simulink model "ZT_VehCtrl_18B_CAN"  (R2018b)
settings: Solver=FixedStepAuto  StartTime=0.0  StopTime=inf  FixedStep=0.005  RelTol=1e-3
InitFcn:
  | mbd_mpc_consistency_checks(bdroot(gcs));
values from neighbouring files (symbols this model uses):
  BatoverTempTh = single(80)    [VCU_INIT.m]
  BRS_PwrValid = single(5)    [VCU_INIT.m]
  BRSEnSpdTh1 = single(10)    [VCU_INIT.m]
  BRSEnSpdTh2 = single(20)    [VCU_INIT.m]
  MCUTempAlarmTh = single (60)    [VCU_INIT.m]
  mps2kmh = single(3.6)    [VCU_INIT.m]
  MtrPwrFac = single(1/9550)    [VCU_INIT.m]
  MtrTempAlarmTh = single (50)    [VCU_INIT.m]
  Padle1Signal1_Th = [PadleSignal1_min,PadleSignal1_max]    [VCU_INIT.m]
  Padle1Signal2_Th = [PadleSignal2_min,PadleSignal2_max]    [VCU_INIT.m]
  PadleSignal1_max = 3.84    [VCU_INIT.m]
  PadleSignal1_min = 0.75    [VCU_INIT.m]
  PadleSignal2_max = 1.92    [VCU_INIT.m]
  PadleSignal2_min = 0.375    [VCU_INIT.m]
  PadleValid = 0.05    [VCU_INIT.m]
  PwrLimFactor = single(0.5)    [VCU_INIT.m]
  Ratio = single(1)    [VCU_INIT.m]
  rpm2mps = single(2*pi/60 * WhlRadius/Ratio)    [VCU_INIT.m]
  SOCLowTh = single(20)    [VCU_INIT.m]
  VehPwrBackwardMax = VehPwrMax * single(0.3)    [VCU_INIT.m]
  VehPwrMax = single(MtrPwrMax * 4)    [VCU_INIT.m]
  VehTrqBackwardMax = VehTrqMax * single(0.3)    [VCU_INIT.m]
  VehTrqMax = single(MtrTrqMax * Ratio *4)    [VCU_INIT.m]
  WhlRadius = single(1)    [VCU_INIT.m]
undefined symbols (not defined in the file or in its folder): Delay_Charge, Delay_Discharge, fifo_0_vect, fifo_1_vect, LQFP, pts1_fifo_0_vect, pts1_fifo_1_vect, pts2_fifo_0_vect, pts2_fifo_1_vect, pts3_fifo_0_vect, pts3_fifo_1_vect, pts4_fifo_0_vect, pts4_fifo_1_vect
libraries: mbd_mpc574x_ec_toolbox x157, canmsglib x74, simulink x38
(part 3 of 12)

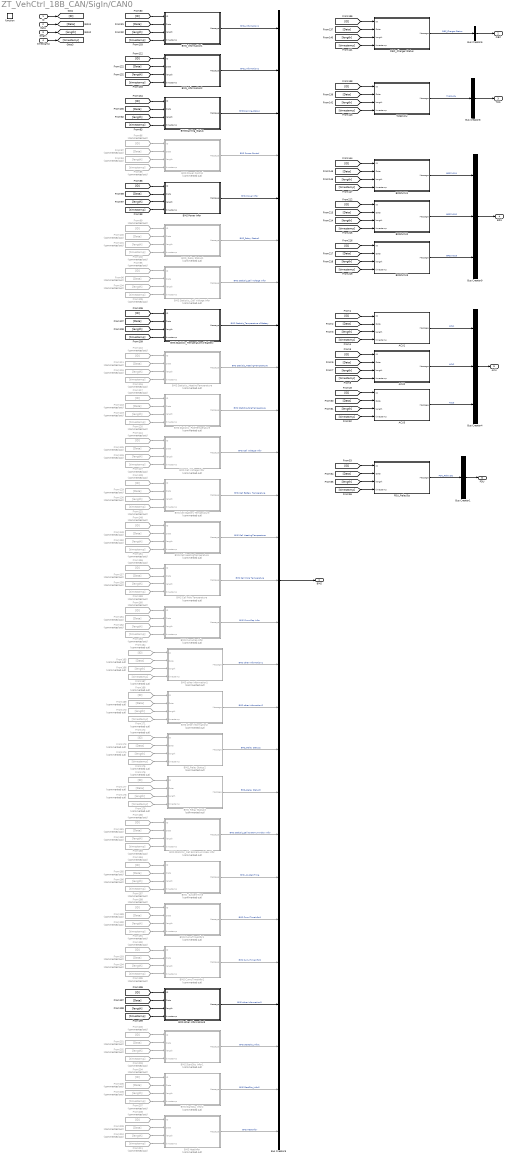
== system ZT_VehCtrl_18B_CAN/SigIn/CAN0  ==
  ID : Inport
  Data : Inport  Port=2
  length : Inport  Port=3
  timestamp : Inport  Port=4
  function : TriggerPort  TriggerType=function-call  VariantControl=Variant
  " BMS Power Control" : Subsystem  Commented=on
  ACU1 : Subsystem
  ACU2 : Subsystem
  ACU3 : Subsystem
  BMS Cell Battery Temperature : Subsystem  Commented=on
  BMS Cell HeatingTemperature : Subsystem  Commented=on
  BMS Cell Pole Temperature : Subsystem  Commented=on
  BMS Cell Voltage Infor : Subsystem  Commented=on
  BMS CumuCap Infor : Subsystem  Commented=on
  BMS CumuTimeInfor1 : Subsystem  Commented=on
  BMS CumuTimeInfor2 : Subsystem  Commented=on
  BMS HeatInfor : Subsystem  Commented=on
  BMS Power Infor : Subsystem
  BMS StartDia_Infor1 : Subsystem  Commented=on
  BMS StartDia_Infor2 : Subsystem  Commented=on
  BMS Statistic_Cell ExtremumIndex Infor : Subsystem  Commented=on
  BMS Statistic_Cell Voltage Infor : Subsystem  Commented=on
  BMS Statistic_HeatingTemperature : Subsystem  Commented=on
  BMS Statistic_PoleTemperature : Subsystem  Commented=on
  BMS Statistic_Temperature of Battery : Subsystem
  "BMS _SystemTime " : Subsystem  Commented=on
  BMS other Information1 : Subsystem  Commented=on
  "BMS other Information2 " : Subsystem  Commented=on
  BMS other Information3 : Subsystem
  BMSWarning_Status : Subsystem
  BMS_Information1 : Subsystem
  BMS_Information2 : Subsystem
  BMS_Relay Status1 : Subsystem  Commented=on
  BMS_Relay Status2 : Subsystem  Commented=on
  BMS_Relay Status3 : Subsystem  Commented=on
  BRS2VCU1 : Subsystem
  BRS2VCU2 : Subsystem
  BRS2VCU3 : Subsystem
  Bus Creator1 : BusCreator  Inputs=1
  Bus Creator4 : BusCreator  Inputs=3
  Bus Creator5 : BusCreator  Inputs=27
  Bus Creator6 : BusCreator  Inputs=1
  Bus Creator8 : BusCreator  Inputs=1
  Bus Creator9 : BusCreator  Inputs=3
  From{87,96,100,111,118,125,129,149,157,161,165,169,173,177,181,185,189,193,201,205,209} (21 alike) : From  Commented=on  GotoTag=Data
  From{84,101,104,115,119,126,130,150,158,162,166,170,174,178,182,186,190,194,202,206,210} (21 alike) : From  Commented=on  GotoTag=length
  From{85,102,105,116,120,127,131,151,159,163,167,171,175,179,183,187,191,195,203,207,211} (21 alike) : From  Commented=on  GotoTag=timestamp
  From{86,95,99,110,117,124,128,148,156,160,164,168,172,176,180,184,188,192,200,204,208} (21 alike) : From  Commented=on  GotoTag=ID
  OBC_Charger Status : Subsystem
  PDU_RelaySts : Subsystem
  TMS2VCU : Subsystem
  BMS : Outport
  OBC : Outport  Port=2
  TMS : Outport  Port=3
  "BRS " : Outport  Port=4
  ACU : Outport  Port=5
  PDU : Outport  Port=6
  wires:
  [timestamp] -> BMS Statistic_Temperature of Battery/4(timestamp)
  From128/1 -> BMS Cell Battery Temperature/1(ID)
  BMS Statistic_PoleTemperature/1(Message) -> Bus Creator5/10  "BMS Statistic_PoleTemperature"
  From100/1 -> BMS_Relay Status1/2(Data)
  BMS Statistic_Temperature of Battery/1(Message) -> Bus Creator5/8  "BMS Statistic_Temperature of Battery"
  BMS Statistic_HeatingTemperature/1(Message) -> Bus Creator5/9  "BMS Statistic_HeatingTemperature"
  From130/1 -> BMS Cell Battery Temperature/3(length)
  From105/1 -> BMS Statistic_Cell Voltage Infor/4(timestamp)
  [length] -> BMS Statistic_Temperature of Battery/3(length)
  BMS Power Infor/1(Message) -> Bus Creator5/5  "BMS Power Infor"
  From131/1 -> BMS Cell Battery Temperature/4(timestamp)
  From117/1 -> BMS Statistic_PoleTemperature/1(ID)
  BMS Cell Battery Temperature/1(Message) -> Bus Creator5/12  "BMS Cell Battery Temperature"
  From96/1 -> BMS Statistic_Cell Voltage Infor/2(Data)
  From119/1 -> BMS Statistic_PoleTemperature/3(length)
  From120/1 -> BMS Statistic_PoleTemperature/4(timestamp)
  From87/1 -> " BMS Power Control"/2(Data)
  From118/1 -> BMS Statistic_PoleTemperature/2(Data)
  From125/1 -> BMS Cell Voltage Infor/2(Data)
  BMS_Relay Status1/1(Message) -> Bus Creator5/6  "BMS_Relay Status1"
  [timestamp] -> BMSWarning_Status/4(timestamp)
  From95/1 -> BMS Statistic_Cell Voltage Infor/1(ID)
  [Data] -> BMS Statistic_Temperature of Battery/2(Data)
  [length] -> BMSWarning_Status/3(length)
  From116/1 -> BMS Statistic_HeatingTemperature/4(timestamp)
  Bus Creator5/1 -> BMS/1
  From85/1 -> " BMS Power Control"/4(timestamp)
  From111/1 -> BMS Statistic_HeatingTemperature/2(Data)
  From86/1 -> " BMS Power Control"/1(ID)
  [Data] -> BMS Power Infor/2(Data)
  BMS Statistic_Cell Voltage Infor/1(Message) -> Bus Creator5/7  "BMS Statistic_Cell Voltage Infor"
  [ID] -> BMSWarning_Status/1(ID)
  From129/1 -> BMS Cell Battery Temperature/2(Data)
  [Data] -> BMSWarning_Status/2(Data)
  From84/1 -> " BMS Power Control"/3(length)
  From124/1 -> BMS Cell Voltage Infor/1(ID)
  BMSWarning_Status/1(Message) -> Bus Creator5/3  "BMSWarning_Status"
  From127/1 -> BMS Cell Voltage Infor/4(timestamp)
  From115/1 -> BMS Statistic_HeatingTemperature/3(length)
  From102/1 -> BMS_Relay Status1/4(timestamp)
  From110/1 -> BMS Statistic_HeatingTemperature/1(ID)
  From104/1 -> BMS Statistic_Cell Voltage Infor/3(length)
  From101/1 -> BMS_Relay Status1/3(length)
  " BMS Power Control"/1(Message) -> Bus Creator5/4  "BMS Power Control"
  [ID] -> BMS Power Infor/1(ID)
  From126/1 -> BMS Cell Voltage Infor/3(length)
  [timestamp] -> BMS Power Infor/4(timestamp)
  [ID] -> BMS Statistic_Temperature of Battery/1(ID)
  BMS Cell Voltage Infor/1(Message) -> Bus Creator5/11  "BMS Cell Voltage Infor"
  From99/1 -> BMS_Relay Status1/1(ID)
  [length] -> BMS Power Infor/3(length)
  [Data] -> OBC_Charger Status/2(Data)
  OBC_Charger Status/1(Message) -> Bus Creator6/1  "OBC_Charger Status"
  [length] -> OBC_Charger Status/3(length)
  [ID] -> OBC_Charger Status/1(ID)
  Bus Creator6/1 -> OBC/1
  [timestamp] -> OBC_Charger Status/4(timestamp)
  BMS_Information2/1(Message) -> Bus Creator5/2  "BMS_Information2"
  BMS_Information1/1(Message) -> Bus Creator5/1  "BMS_Information1"
  [ID] -> BMS_Information2/1(ID)
  [Data] -> BMS_Information2/2(Data)
  [length] -> BMS_Information2/3(length)
  [timestamp] -> BMS_Information1/4(timestamp)
  [length] -> BMS_Information1/3(length)
  [Data] -> BMS_Information1/2(Data)
  [ID] -> BMS_Information1/1(ID)
  [timestamp] -> BMS_Information2/4(timestamp)
  From149/1 -> BMS Cell HeatingTemperature/2(Data)
  BMS Cell HeatingTemperature/1(Message) -> Bus Creator5/13  "BMS Cell HeatingTemperature"
  From151/1 -> BMS Cell HeatingTemperature/4(timestamp)
  From150/1 -> BMS Cell HeatingTemperature/3(length)
  From148/1 -> BMS Cell HeatingTemperature/1(ID)
  From156/1 -> BMS Cell Pole Temperature/1(ID)
  From158/1 -> BMS Cell Pole Temperature/3(length)
  From159/1 -> BMS Cell Pole Temperature/4(timestamp)
  BMS Cell Pole Temperature/1(Message) -> Bus Creator5/14  "BMS Cell Pole Temperature"
  From157/1 -> BMS Cell Pole Temperature/2(Data)
  From161/1 -> BMS CumuCap Infor/2(Data)
  BMS CumuCap Infor/1(Message) -> Bus Creator5/15  "BMS CumuCap Infor"
  From163/1 -> BMS CumuCap Infor/4(timestamp)
  From162/1 -> BMS CumuCap Infor/3(length)
  From160/1 -> BMS CumuCap Infor/1(ID)
  From164/1 -> BMS other Information1/1(ID)
  From166/1 -> BMS other Information1/3(length)
  From167/1 -> BMS other Information1/4(timestamp)
  BMS other Information1/1(Message) -> Bus Creator5/16  "BMS other Information1"
  From165/1 -> BMS other Information1/2(Data)
  From169/1 -> "BMS other Information2 "/2(Data)
  "BMS other Information2 "/1(Message) -> Bus Creator5/17  "BMS other Information2"
  From171/1 -> "BMS other Information2 "/4(timestamp)
  From170/1 -> "BMS other Information2 "/3(length)
  From168/1 -> "BMS other Information2 "/1(ID)
  From172/1 -> BMS_Relay Status2/1(ID)
  From174/1 -> BMS_Relay Status2/3(length)
  From175/1 -> BMS_Relay Status2/4(timestamp)
  BMS_Relay Status2/1(Message) -> Bus Creator5/18  "BMS_Relay Status2"
  From173/1 -> BMS_Relay Status2/2(Data)
  From177/1 -> BMS_Relay Status3/2(Data)
  BMS_Relay Status3/1(Message) -> Bus Creator5/19  "BMS_Relay Status3"
  From179/1 -> BMS_Relay Status3/4(timestamp)
  From178/1 -> BMS_Relay Status3/3(length)
  From176/1 -> BMS_Relay Status3/1(ID)
  From180/1 -> BMS Statistic_Cell ExtremumIndex Infor/1(ID)
  From182/1 -> BMS Statistic_Cell ExtremumIndex Infor/3(length)
  From183/1 -> BMS Statistic_Cell ExtremumIndex Infor/4(timestamp)
  BMS Statistic_Cell ExtremumIndex Infor/1(Message) -> Bus Creator5/20  "BMS Statistic_Cell ExtremumIndex Infor"
  From181/1 -> BMS Statistic_Cell ExtremumIndex Infor/2(Data)
  From185/1 -> "BMS _SystemTime "/2(Data)
  "BMS _SystemTime "/1(Message) -> Bus Creator5/21  "BMS _SystemTime"
  From187/1 -> "BMS _SystemTime "/4(timestamp)
  From186/1 -> "BMS _SystemTime "/3(length)
  From184/1 -> "BMS _SystemTime "/1(ID)
  From188/1 -> BMS CumuTimeInfor1/1(ID)
  From190/1 -> BMS CumuTimeInfor1/3(length)
  From191/1 -> BMS CumuTimeInfor1/4(timestamp)
  BMS CumuTimeInfor1/1(Message) -> Bus Creator5/22  "BMS CumuTimeInfor1"
  From189/1 -> BMS CumuTimeInfor1/2(Data)
  From193/1 -> BMS CumuTimeInfor2/2(Data)
  BMS CumuTimeInfor2/1(Message) -> Bus Creator5/23  "BMS CumuTimeInfor2"
  From195/1 -> BMS CumuTimeInfor2/4(timestamp)
  From194/1 -> BMS CumuTimeInfor2/3(length)
  From192/1 -> BMS CumuTimeInfor2/1(ID)
  [ID] -> BMS other Information3/1(ID)
  [length] -> BMS other Information3/3(length)
  [timestamp] -> BMS other Information3/4(timestamp)
  BMS other Information3/1(Message) -> Bus Creator5/24  "BMS other Information3"
  [Data] -> BMS other Information3/2(Data)
  From201/1 -> BMS StartDia_Infor1/2(Data)
  BMS StartDia_Infor1/1(Message) -> Bus Creator5/25  "BMS StartDia_Infor1"
  From203/1 -> BMS StartDia_Infor1/4(timestamp)
  From202/1 -> BMS StartDia_Infor1/3(length)
  From200/1 -> BMS StartDia_Infor1/1(ID)
  From204/1 -> BMS StartDia_Infor2/1(ID)
  From206/1 -> BMS StartDia_Infor2/3(length)
  From207/1 -> BMS StartDia_Infor2/4(timestamp)
  BMS StartDia_Infor2/1(Message) -> Bus Creator5/26  "BMS StartDia_Infor2"
  From205/1 -> BMS StartDia_Infor2/2(Data)
  From209/1 -> BMS HeatInfor/2(Data)
  BMS HeatInfor/1(Message) -> Bus Creator5/27  "BMS HeatInfor"
  From211/1 -> BMS HeatInfor/4(timestamp)
  From210/1 -> BMS HeatInfor/3(length)
  From208/1 -> BMS HeatInfor/1(ID)
  [timestamp] -> TMS2VCU/4(timestamp)
  Bus Creator8/1 -> TMS/1
  [ID] -> TMS2VCU/1(ID)
  [length] -> TMS2VCU/3(length)
  TMS2VCU/1(Message) -> Bus Creator8/1  "TMS2VCU"
  [Data] -> TMS2VCU/2(Data)
  [Data] -> BRS2VCU1/2(Data)
  BRS2VCU1/1(Message) -> Bus Creator9/1  "BRS2VCU1"
  [length] -> BRS2VCU1/3(length)
  [ID] -> BRS2VCU1/1(ID)
  Bus Creator9/1 -> "BRS "/1
  [timestamp] -> BRS2VCU1/4(timestamp)
  [timestamp] -> BRS2VCU2/4(timestamp)
  [ID] -> BRS2VCU2/1(ID)
  [length] -> BRS2VCU2/3(length)
  [Data] -> BRS2VCU2/2(Data)
  [Data] -> BRS2VCU3/2(Data)
  [length] -> BRS2VCU3/3(length)
  [ID] -> BRS2VCU3/1(ID)
  [timestamp] -> BRS2VCU3/4(timestamp)
  BRS2VCU2/1(Message) -> Bus Creator9/2  "BRS2VCU2"
  BRS2VCU3/1(Message) -> Bus Creator9/3  "BRS2VCU3"
  length/1 -> [length]
  ID/1 -> [ID]
  timestamp/1 -> [timestamp]
  Data/1 -> [Data]
  [Data] -> ACU1/2(Data)
  [timestamp] -> ACU1/4(timestamp)
  [length] -> ACU2/3(length)
  [timestamp] -> ACU3/4(timestamp)
  [ID] -> ACU3/1(ID)
  ACU2/1(Message) -> Bus Creator4/2  "ACU2"
  Bus Creator4/1 -> ACU/1
  [Data] -> ACU2/2(Data)
  [length] -> ACU1/3(length)
  [timestamp] -> ACU2/4(timestamp)
  [ID] -> ACU1/1(ID)
  [length] -> ACU3/3(length)
  ACU1/1(Message) -> Bus Creator4/1  "ACU1"
  ACU3/1(Message) -> Bus Creator4/3  "ACU3"
  [Data] -> ACU3/2(Data)
  [ID] -> ACU2/1(ID)
  Bus Creator1/1 -> PDU/1
  [length] -> PDU_RelaySts/3(length)
  PDU_RelaySts/1(Message) -> Bus Creator1/1  "PDU_RelaySts"
  [Data] -> PDU_RelaySts/2(Data)
  [timestamp] -> PDU_RelaySts/4(timestamp)
  [ID] -> PDU_RelaySts/1(ID)

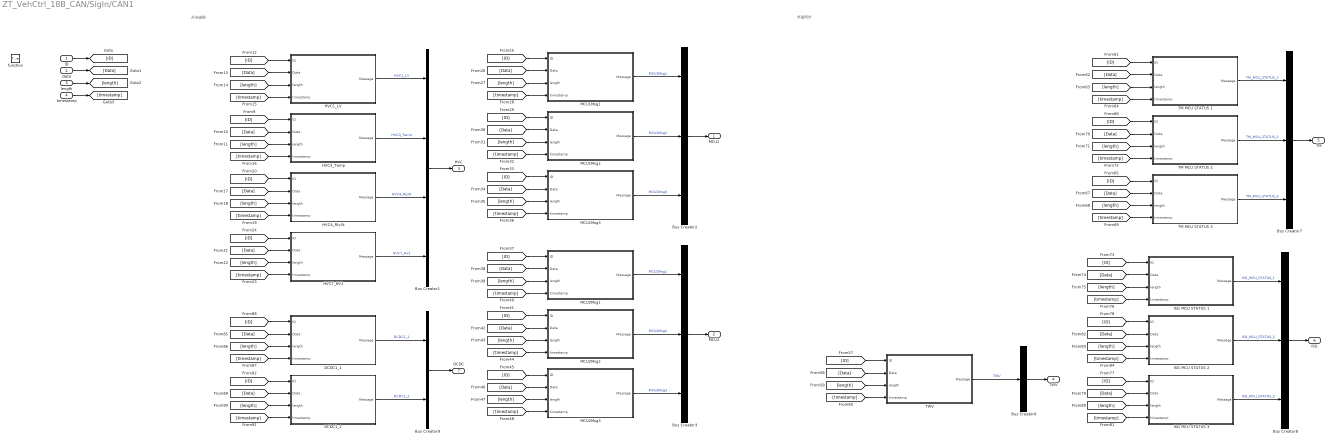
== system ZT_VehCtrl_18B_CAN/SigIn/CAN1 ==
  note: 永磁同步
  note: 开关磁阻
  ID : Inport
  Data : Inport  Port=2
  length : Inport  Port=3
  timestamp : Inport  Port=4
  function : TriggerPort  TriggerType=function-call  VariantControl=Variant
  Bus Creator1 : BusCreator  Inputs=4
  Bus Creator{2..3,7..8} (4 alike) : BusCreator  Inputs=3
  Bus Creator6 : BusCreator  Inputs=1
  Bus Creator9 : BusCreator  Inputs=2
  DCDC1_1 : Subsystem
  DCDC1_2 : Subsystem
  HVC1_LV : Subsystem
  HVC3_Temp : Subsystem
  HVC4_RlySt : Subsystem
  HVC7_HV1 : Subsystem
  ISG MCU STATUS 1 : Subsystem
  ISG MCU STATUS 2 : Subsystem
  ISG MCU STATUS 3 : Subsystem
  MCU1Msg1 : Subsystem
  MCU1Msg2 : Subsystem
  MCU1Msg3 : Subsystem
  MCU2Msg1 : Subsystem
  MCU2Msg2 : Subsystem
  MCU2Msg3 : Subsystem
  TM MCU STATUS 1 : Subsystem
  TM MCU STATUS 2 : Subsystem
  TM MCU STATUS 3 : Subsystem
  "TWV " : Subsystem
  MCU1 : Outport
  MCU2 : Outport  Port=2
  HVC : Outport  Port=3
  TWV : Outport  Port=4
  TM : Outport  Port=5
  "ISG " : Outport  Port=6
  DCDC : Outport  Port=7
  wires:
  length/1 -> [length]
  timestamp/1 -> [timestamp]
  Data/1 -> [Data]
  ID/1 -> [ID]
  Bus Creator2/1 -> MCU1/1
  [Data] -> HVC1_LV/2(Data)
  [timestamp] -> HVC1_LV/4(timestamp)
  [ID] -> HVC1_LV/1(ID)
  HVC1_LV/1(Message) -> Bus Creator1/1  "HVC1_LV"
  [length] -> HVC1_LV/3(length)
  [length] -> HVC3_Temp/3(length)
  HVC3_Temp/1(Message) -> Bus Creator1/2  "HVC3_Temp"
  [ID] -> HVC3_Temp/1(ID)
  [timestamp] -> HVC3_Temp/4(timestamp)
  [Data] -> HVC3_Temp/2(Data)
  [Data] -> HVC4_RlySt/2(Data)
  [timestamp] -> HVC4_RlySt/4(timestamp)
  [ID] -> HVC4_RlySt/1(ID)
  [length] -> HVC4_RlySt/3(length)
  HVC4_RlySt/1(Message) -> Bus Creator1/3  "HVC4_RlySt"
  HVC7_HV1/1(Message) -> Bus Creator1/4  "HVC7_HV1"
  [length] -> HVC7_HV1/3(length)
  [ID] -> HVC7_HV1/1(ID)
  [timestamp] -> HVC7_HV1/4(timestamp)
  [Data] -> HVC7_HV1/2(Data)
  [length] -> MCU1Msg1/3(length)
  MCU1Msg1/1(Message) -> Bus Creator2/1  "MCU1Msg1"
  [ID] -> MCU1Msg1/1(ID)
  [timestamp] -> MCU1Msg1/4(timestamp)
  [Data] -> MCU1Msg1/2(Data)
  [Data] -> MCU1Msg2/2(Data)
  [timestamp] -> MCU1Msg2/4(timestamp)
  [ID] -> MCU1Msg2/1(ID)
  MCU1Msg2/1(Message) -> Bus Creator2/2  "MCU1Msg2"
  [length] -> MCU1Msg2/3(length)
  [length] -> MCU1Msg3/3(length)
  [ID] -> MCU1Msg3/1(ID)
  [timestamp] -> MCU1Msg3/4(timestamp)
  [Data] -> MCU1Msg3/2(Data)
  MCU1Msg3/1(Message) -> Bus Creator2/3  "MCU1Msg3"
  MCU2Msg3/1(Message) -> Bus Creator3/3  "MCU2Msg3"
  [Data] -> MCU2Msg3/2(Data)
  [timestamp] -> MCU2Msg3/4(timestamp)
  [ID] -> MCU2Msg3/1(ID)
  [length] -> MCU2Msg3/3(length)
  [length] -> MCU2Msg2/3(length)
  MCU2Msg2/1(Message) -> Bus Creator3/2  "MCU2Msg2"
  [ID] -> MCU2Msg2/1(ID)
  [timestamp] -> MCU2Msg2/4(timestamp)
  [Data] -> MCU2Msg2/2(Data)
  [Data] -> MCU2Msg1/2(Data)
  [timestamp] -> MCU2Msg1/4(timestamp)
  [ID] -> MCU2Msg1/1(ID)
  MCU2Msg1/1(Message) -> Bus Creator3/1  "MCU2Msg1"
  [length] -> MCU2Msg1/3(length)
  Bus Creator6/1 -> TWV/1
  "TWV "/1(Message) -> Bus Creator6/1  "TWV"
  [Data] -> "TWV "/2(Data)
  [timestamp] -> "TWV "/4(timestamp)
  [ID] -> "TWV "/1(ID)
  [length] -> "TWV "/3(length)
  Bus Creator7/1 -> TM/1
  [length] -> TM MCU STATUS 1/3(length)
  TM MCU STATUS 1/1(Message) -> Bus Creator7/1  "TM_MCU_STATUS_1"
  [ID] -> TM MCU STATUS 1/1(ID)
  [timestamp] -> TM MCU STATUS 1/4(timestamp)
  [Data] -> TM MCU STATUS 1/2(Data)
  [Data] -> TM MCU STATUS 2/2(Data)
  [timestamp] -> TM MCU STATUS 2/4(timestamp)
  [ID] -> TM MCU STATUS 2/1(ID)
  TM MCU STATUS 2/1(Message) -> Bus Creator7/2  "TM_MCU_STATUS_2"
  [length] -> TM MCU STATUS 2/3(length)
  [length] -> TM MCU STATUS 3/3(length)
  [ID] -> TM MCU STATUS 3/1(ID)
  [timestamp] -> TM MCU STATUS 3/4(timestamp)
  [Data] -> TM MCU STATUS 3/2(Data)
  TM MCU STATUS 3/1(Message) -> Bus Creator7/3  "TM_MCU_STATUS_3"
  ISG MCU STATUS 3/1(Message) -> Bus Creator8/3  "ISG_MCU_STATUS_3"
  [Data] -> ISG MCU STATUS 3/2(Data)
  [timestamp] -> ISG MCU STATUS 3/4(timestamp)
  [ID] -> ISG MCU STATUS 3/1(ID)
  [length] -> ISG MCU STATUS 3/3(length)
  [length] -> ISG MCU STATUS 2/3(length)
  ISG MCU STATUS 2/1(Message) -> Bus Creator8/2  "ISG_MCU_STATUS_2"
  [ID] -> ISG MCU STATUS 2/1(ID)
  [timestamp] -> ISG MCU STATUS 2/4(timestamp)
  [Data] -> ISG MCU STATUS 2/2(Data)
  [Data] -> ISG MCU STATUS 1/2(Data)
  [timestamp] -> ISG MCU STATUS 1/4(timestamp)
  [ID] -> ISG MCU STATUS 1/1(ID)
  ISG MCU STATUS 1/1(Message) -> Bus Creator8/1  "ISG_MCU_STATUS_1"
  [length] -> ISG MCU STATUS 1/3(length)
  Bus Creator8/1 -> "ISG "/1
  Bus Creator1/1 -> HVC/1
  Bus Creator3/1 -> MCU2/1
  [Data] -> DCDC1_2/2(Data)
  [timestamp] -> DCDC1_2/4(timestamp)
  [ID] -> DCDC1_2/1(ID)
  [length] -> DCDC1_2/3(length)
  DCDC1_2/1(Message) -> Bus Creator9/2  "DCDC1_2"
  DCDC1_1/1(Message) -> Bus Creator9/1  "DCDC1_1"
  [length] -> DCDC1_1/3(length)
  [ID] -> DCDC1_1/1(ID)
  [timestamp] -> DCDC1_1/4(timestamp)
  [Data] -> DCDC1_1/2(Data)
  Bus Creator9/1 -> DCDC/1

== system ZT_VehCtrl_18B_CAN/SigIn/DI ==
  note: DI PULLDOWN
  note: DI PULLUP
  Bus Creator : BusCreator  Inputs=14
  DI01 : mbd_mpc574x_ec_toolbox/GPIO Blocks/Digital_Input  gpio_pin=PTG5: [SIUL2_GPIO101 | General Purpose IO PG[5]]  pull_resistor=None
  DI02 : mbd_mpc574x_ec_toolbox/GPIO Blocks/Digital_Input  gpio_pin=PTG9: [SIUL2_GPIO105 | General Purpose IO PG[9]]  pull_resistor=None
  DI03 : mbd_mpc574x_ec_toolbox/GPIO Blocks/Digital_Input  gpio_pin=PTC11: [SIUL2_GPIO43 | General Purpose IO PC[11]]  pull_resistor=None
  DI04 : mbd_mpc574x_ec_toolbox/GPIO Blocks/Digital_Input  gpio_pin=PTA9: [SIUL2_GPIO9 | General Purpose IO PA[9]]  pull_resistor=None
  DI07 : mbd_mpc574x_ec_toolbox/GPIO Blocks/Digital_Input  gpio_pin=PTA0: [SIUL2_GPIO0 | General Purpose IO PA[0]]  pull_resistor=None
  DI08 : mbd_mpc574x_ec_toolbox/GPIO Blocks/Digital_Input  gpio_pin=PTD11: [SIUL2_GPIO59 | General Purpose IO PD[11]]  pull_resistor=None
  DI09 : mbd_mpc574x_ec_toolbox/GPIO Blocks/Digital_Input  gpio_pin=PTG6: [SIUL2_GPIO102 | General Purpose IO PG[6]]  pull_resistor=None
  DI10 : mbd_mpc574x_ec_toolbox/GPIO Blocks/Digital_Input  gpio_pin=PTG2: [SIUL2_GPIO98 | General Purpose IO PG[2]]  pull_resistor=None
  DI12 : mbd_mpc574x_ec_toolbox/GPIO Blocks/Digital_Input  gpio_pin=PTF13: [SIUL2_GPIO93 | General Purpose IO PF[13]]  pull_resistor=None
  DI13 : mbd_mpc574x_ec_toolbox/GPIO Blocks/Digital_Input  gpio_pin=PTG4: [SIUL2_GPIO100 | General Purpose IO PG[4]]  pull_resistor=None
  DI15 : mbd_mpc574x_ec_toolbox/GPIO Blocks/Digital_Input  gpio_pin=PTF12: [SIUL2_GPIO92 | General Purpose IO PF[12]]  pull_resistor=None
  DI16 : mbd_mpc574x_ec_toolbox/GPIO Blocks/Digital_Input  gpio_pin=PTG7: [SIUL2_GPIO103 | General Purpose IO PG[7]]  pull_resistor=None
  DI17 : mbd_mpc574x_ec_toolbox/GPIO Blocks/Digital_Input  gpio_pin=PTD10: [SIUL2_GPIO58 | General Purpose IO PD[10]]  pull_resistor=None
  DI18 : mbd_mpc574x_ec_toolbox/GPIO Blocks/Digital_Input  gpio_pin=PTG10: [SIUL2_GPIO106 | General Purpose IO PG[10]]  pull_resistor=None
  DI_31_32_33_34 : Subsystem
  Data Store Read : DataStoreRead  DataStoreName=DI07
  Data Store Read1 : DataStoreRead  DataStoreName=DI10
  Data Store Read10 : DataStoreRead  DataStoreName=DI04
  Data Store Read11 : DataStoreRead  DataStoreName=DI12
  Data Store Read12 : DataStoreRead  DataStoreName=DI08
  Data Store Read13 : DataStoreRead  DataStoreName=DI09
  Data Store Read2 : DataStoreRead  DataStoreName=DI13
  Data Store Read3 : DataStoreRead  DataStoreName=DI15
  Data Store Read4 : DataStoreRead  DataStoreName=DI16
  Data Store Read5 : DataStoreRead  DataStoreName=DI17
  Data Store Read6 : DataStoreRead  DataStoreName=DI18
  Data Store Read7 : DataStoreRead  DataStoreName=DI01
  Data Store Read8 : DataStoreRead  DataStoreName=DI02
  Data Store Read9 : DataStoreRead  DataStoreName=DI03
  Data Store Write : DataStoreWrite  DataStoreName=DI07
  Data Store Write1 : DataStoreWrite  DataStoreName=DI01
  Data Store Write10 : DataStoreWrite  DataStoreName=DI04
  Data Store Write11 : DataStoreWrite  DataStoreName=DI12
  Data Store Write12 : DataStoreWrite  DataStoreName=DI08
  Data Store Write13 : DataStoreWrite  DataStoreName=DI09
  Data Store Write2 : DataStoreWrite  DataStoreName=DI10
  Data Store Write3 : DataStoreWrite  DataStoreName=DI13
  Data Store Write4 : DataStoreWrite  DataStoreName=DI15
  Data Store Write5 : DataStoreWrite  DataStoreName=DI16
  Data Store Write6 : DataStoreWrite  DataStoreName=DI17
  Data Store Write7 : DataStoreWrite  DataStoreName=DI18
  Data Store Write8 : DataStoreWrite  DataStoreName=DI02
  Data Store Write9 : DataStoreWrite  DataStoreName=DI03
  DI : Outport
  wires:
  DI07/1 -> Data Store Write/1
  DI01/1 -> Data Store Write1/1
  DI10/1 -> Data Store Write2/1
  DI13/1 -> Data Store Write3/1
  DI15/1 -> Data Store Write4/1
  DI17/1 -> Data Store Write6/1
  DI16/1 -> Data Store Write5/1
  DI18/1 -> Data Store Write7/1
  DI09/1 -> Data Store Write13/1
  DI08/1 -> Data Store Write12/1
  DI12/1 -> Data Store Write11/1
  DI04/1 -> Data Store Write10/1
  DI02/1 -> Data Store Write8/1
  DI03/1 -> Data Store Write9/1
  Data Store Read/1 -> Bus Creator/1  "DI07"
  Data Store Read1/1 -> Bus Creator/2  "DI10"
  Data Store Read2/1 -> Bus Creator/3  "DI13"
  Data Store Read3/1 -> Bus Creator/4  "DI15"
  Data Store Read4/1 -> Bus Creator/5  "DI16"
  Data Store Read5/1 -> Bus Creator/6  "DI17"
  Data Store Read6/1 -> Bus Creator/7  "DI18"
  Data Store Read7/1 -> Bus Creator/8  "DI01"
  Data Store Read8/1 -> Bus Creator/9  "DI02"
  Data Store Read9/1 -> Bus Creator/10  "DI03"
  Data Store Read10/1 -> Bus Creator/11  "DI04"
  Data Store Read11/1 -> Bus Creator/12  "DI12"
  Data Store Read12/1 -> Bus Creator/13  "DI08"
  Data Store Read13/1 -> Bus Creator/14  "DI09"
  Bus Creator/1 -> DI/1

== system ZT_VehCtrl_18B_CAN/SigIn/PWM ==
  note: DI PWM PULLDOWN
  note: DI PWM PULLUP
  Bus Creator : BusCreator  Inputs=8
  Data Store Read : DataStoreRead  DataStoreName=DI31_PWM_DC
  Data Store Read1 : DataStoreRead  DataStoreName=DI31_PWM_FRQ
  Data Store Read2 : DataStoreRead  DataStoreName=DI32_PWM_DC
  Data Store Read3 : DataStoreRead  DataStoreName=DI32_PWM_FRQ
  Data Store Read4 : DataStoreRead  DataStoreName=DI33_PWM_DC
  Data Store Read5 : DataStoreRead  DataStoreName=DI33_PWM_FRQ
  Data Store Read6 : DataStoreRead  DataStoreName=DI34_PWM_DC
  Data Store Read7 : DataStoreRead  DataStoreName=DI34_PWM_FRQ
  Data Store Write : DataStoreWrite  DataStoreName=DI31_PWM_DC
  Data Store Write1 : DataStoreWrite  DataStoreName=DI31_PWM_FRQ
  Data Store Write2 : DataStoreWrite  DataStoreName=DI32_PWM_DC
  Data Store Write3 : DataStoreWrite  DataStoreName=DI32_PWM_FRQ
  Data Store Write4 : DataStoreWrite  DataStoreName=DI33_PWM_DC
  Data Store Write5 : DataStoreWrite  DataStoreName=DI33_PWM_FRQ
  Data Store Write6 : DataStoreWrite  DataStoreName=DI34_PWM_FRQ
  Data Store Write7 : DataStoreWrite  DataStoreName=DI34_PWM_DC
  PWM_PTS1 : Subsystem
  PWM_PTS2 : Subsystem
  PWM_PTS3 : Subsystem
  PWM_PTS4 : Subsystem
  Subsystem : Subsystem  Commented=on
  eTimer_Arm_Capture : mbd_mpc574x_ec_toolbox/Motor Control Blocks/eTIMER Blocks/eTimer_Arm_Capture  etimerModule=0  etimerChannel=2  etimerArmAction=Start
  eTimer_Arm_Capture1 : mbd_mpc574x_ec_toolbox/Motor Control Blocks/eTIMER Blocks/eTimer_Arm_Capture  etimerModule=1  etimerChannel=2  etimerArmAction=Start
  eTimer_Arm_Capture2 : mbd_mpc574x_ec_toolbox/Motor Control Blocks/eTIMER Blocks/eTimer_Arm_Capture  etimerModule=1  etimerChannel=1  etimerArmAction=Start
  eTimer_Arm_Capture3 : mbd_mpc574x_ec_toolbox/Motor Control Blocks/eTIMER Blocks/eTimer_Arm_Capture  etimerModule=1  etimerChannel=3  etimerArmAction=Start
  PWMIn : Outport
  wires:
  Bus Creator/1 -> PWMIn/1
  Data Store Read7/1 -> Bus Creator/8  "DI34_PWM_FRQ"
  Data Store Read6/1 -> Bus Creator/7  "DI34_PWM_DC"
  Data Store Read5/1 -> Bus Creator/6  "DI33_PWM_FRQ"
  Data Store Read4/1 -> Bus Creator/5  "DI33_PWM_DC"
  Data Store Read3/1 -> Bus Creator/4  "DI32_PWM_FRQ"
  Data Store Read2/1 -> Bus Creator/3  "DI32_PWM_DC"
  Data Store Read1/1 -> Bus Creator/2  "DI31_PWM_FRQ"
  Data Store Read/1 -> Bus Creator/1  "DI31_PWM_DC"
  PWM_PTS4/1(DC) -> Data Store Write/1
  PWM_PTS4/2(freq) -> Data Store Write1/1
  PWM_PTS1/1(DC) -> Data Store Write2/1
  PWM_PTS1/2(freq) -> Data Store Write3/1
  PWM_PTS2/1(DC) -> Data Store Write4/1
  PWM_PTS2/2(freq) -> Data Store Write5/1
  PWM_PTS3/2(freq) -> Data Store Write6/1
  PWM_PTS3/1(DC) -> Data Store Write7/1

== system ZT_VehCtrl_18B_CAN/SigIn/Subsystem ==
  AI08 : Inport
  AI12 : Inport  Port=2
  1-D Lookup Table : Lookup_n-D  NumberOfTableDimensions=1  BreakpointsForDimension1=Padle1Signal1_Th  Table=[0,1]  InternalRulePriority=Speed  RndMeth=Simplest  InputSameDT=on
  1-D Lookup Table1 : Lookup_n-D  NumberOfTableDimensions=1  BreakpointsForDimension1=Padle1Signal2_Th  Table=[0,1]  InternalRulePriority=Speed  RndMeth=Simplest  InputSameDT=on
  Abs : Abs
  Compare To Constant : simulink/Logic and Bit Operations/Compare To Constant  relop=<=  const=PadleValid  OutDataTypeStr=boolean
  Constant2 : Constant  Value=0  OutDataTypeStr=single
  Data Type Conversion : DataTypeConversion  OutDataTypeStr=single
  Data Type Conversion1 : DataTypeConversion  OutDataTypeStr=single
  Saturation : Saturate  UpperLimit=PadleSignal1_max  LowerLimit=PadleSignal1_min
  Saturation1 : Saturate  UpperLimit=PadleSignal2_max  LowerLimit=PadleSignal2_min  LinearizeAsGain=off
  Subtract : Sum  Inputs=+-
  Switch : Switch  Criteria=u2 > Threshold
  "ACCPadle " : Outport
  wires:
  Subtract/1 -> Abs/1
  Saturation/1 -> 1-D Lookup Table/1
  Saturation1/1 -> 1-D Lookup Table1/1
  1-D Lookup Table/1 -> Data Type Conversion/1, Subtract/1
  Switch/1 -> Data Type Conversion1/1
  Constant2/1 -> Switch/3
  1-D Lookup Table1/1 -> Subtract/2
  Data Type Conversion/1 -> Switch/1
  Compare To Constant/1 -> Switch/2
  Abs/1 -> Compare To Constant/1
  AI08/1 -> Saturation/1
  AI12/1 -> Saturation1/1
  Data Type Conversion1/1 -> "ACCPadle "/1

== system ZT_VehCtrl_18B_CAN/SigOut/ACU ==
  "ACU_OUT " : Inport
  Trigger : TriggerPort  VariantControl=Variant  PortDimensions=1
  Add : Sum
  Bus Selector : BusSelector  OutputSignals=Data,Length
  Bus Selector1 : BusSelector  Commented=on  OutputSignals=DcacEpsCmd,DcdcCmd
  Constant : Constant  OutDataTypeStr=uint8
  Constant1 : Constant  Commented=on  Value=85
  Constant2 : Constant  Commented=on  Value=170
  Data Store Read : DataStoreRead  DataStoreName=Cnt_ACU_OUT
  Data Store Read1 : DataStoreRead  DataStoreName=DcdcCmd
  Data Store Read2 : DataStoreRead  DataStoreName=DcacEpsCmd
  Data Store Read3 : DataStoreRead  DataStoreName=DcacEpsMode
  Data Store Read4 : DataStoreRead  DataStoreName=DcacAcCmd
  Data Store Write : DataStoreWrite  DataStoreName=Cnt_ACU_OUT
  Data Type Conversion{,1..3} (4 alike) : DataTypeConversion  OutDataTypeStr=single
  FCAN_Send_ID_0x0C079AA7 : mbd_mpc574x_ec_toolbox/Communication Blocks/CAN Blocks/FCAN_Send  Priority=2  can_instance=0  can_mode=Non-blocking  can_timeout_ms=0  can_mb_idx=51  can_extended_id=on  can_is_remote=off  can_id=0C079AA7  show_adv_opts=off  can_fd_enable=off  can_enable_brs=off  can_fd_padding=0
      settings: SourceProductName=NXP Model-Based Design Toolbox for MPC57xx MCUs
  Subsystem1 : Subsystem
  Subsystem2 : Subsystem
  Subsystem3 : Subsystem
  Subsystem4 : Subsystem
  VCU_ACU1 : canmsglib/CAN Pack  CANdbFile=D:\VCU\VCU_SL_ZhengZhou\ZT2\模型与接口\CAN_DBC\动力CANB_GBK.dbc  MsgList=(none)  MsgName=VCU_ACU1  MsgIDType=Extended (29-bit identifier)  MsgIdentifier=201824935  MsgLength=8  SignalInfo=DcacAcCmd$32$8$1$2$1$0$1$0$-Inf$Inf$#DcacEpsCmd$16$8$1$2$1$0$1$0$-Inf$Inf$#DcacEpsMode$24$8$1$2$1$0$1$0$-Inf$Inf$#DcdcCmd$0$8$1$2$1$0$1$0$-Inf$Inf$#  NSignals=4  StartBits=str2num('[int32(32);int32(16);int32(24);int32(0)]')  SignalSizes=str2num('[int32(8);int32(8);int32(8);int32(8)]')  ByteOrders=str2num('[int32(1);int32(1);int32(1);int32(1)]')  DataTypes=str2num('[int32(2);int32(2);int32(2);int32(2)]')  MultiplexTypes=str2num('[int32(1);int32(1);int32(1);int32(1)]')  MultiplexValues=str2num('[double(0);double(0);double(0);double(0)]')  Factors=str2num('[double(1);double(1);double(1);double(1)]')  Offsets=str2num('[double(0);double(0);double(0);double(0)]')  Minimums=str2num('[double(-Inf);double(-Inf);double(-Inf);double(-Inf)]')  Maximums=str2num('[double(Inf);double(Inf);double(Inf);double(Inf)]')  Remote=off  ApplyMinMax=off  BusOutput=on
      settings: SourceProductName=Simulink Real-Time  SourceProductBaseCode=XP  DataFormat=CANdb specified signals
  wires:
  VCU_ACU1/1 -> Bus Selector/1
  Bus Selector/2 -> FCAN_Send_ID_0x0C079AA7/2  "<Length>"
  Bus Selector/1 -> FCAN_Send_ID_0x0C079AA7/1  "<Data>"
  Add/1 -> Data Store Write/1
  Data Store Read/1 -> Add/1
  Constant/1 -> Add/2
  "ACU_OUT "/1 -> Bus Selector1/1
  Bus Selector1/1 -> ?  "<DcacEpsCmd>"
  Bus Selector1/2 -> ?  "<DcdcCmd>"
  Subsystem1/1(Out1) -> Data Type Conversion/1
  Subsystem3/1(Out1) -> Data Type Conversion2/1
  Constant1/1 -> ?
  Constant2/1 -> ?
  Data Store Read1/1 -> Subsystem1/1(<DcacEpsCmd>)
  Data Store Read3/1 -> Subsystem2/1(<DcacEpsCmd>)
  Data Store Read2/1 -> Subsystem3/1(<DcacEpsCmd>)
  Data Store Read4/1 -> Subsystem4/1(<DcacEpsCmd>)
  Subsystem2/1(Out1) -> Data Type Conversion1/1
  Subsystem4/1(Out1) -> Data Type Conversion3/1
  Data Type Conversion/1 -> VCU_ACU1/4
  Data Type Conversion1/1 -> VCU_ACU1/3
  Data Type Conversion2/1 -> VCU_ACU1/2
  Data Type Conversion3/1 -> VCU_ACU1/1

== system ZT_VehCtrl_18B_CAN/SigOut/BMS ==
  "BMS_OUT " : Inport
  Trigger : TriggerPort  VariantControl=Variant  PortDimensions=1
  Add : Sum
  Bus Selector : BusSelector  OutputSignals=Data,Length
  Bus Selector1 : BusSelector  Commented=on  OutputSignals=VCU_PowerOnReq,VCU_UrgencyCutOffPowerReq
  Constant2 : Constant  OutDataTypeStr=uint8
  Data Store Read : DataStoreRead  DataStoreName=Cnt_BMS_OUT
  Data Store Read1 : DataStoreRead  DataStoreName=VCU_PowerOnReq
  Data Store Read2 : DataStoreRead  DataStoreName=VCU_UrgencyCutOffPowerReq
  Data Store Write : DataStoreWrite  DataStoreName=Cnt_BMS_OUT
  Data Type Conversion : DataTypeConversion  OutDataTypeStr=boolean
  Data Type Conversion1 : DataTypeConversion  OutDataTypeStr=boolean
  FCAN_Send_ID_0x160 : mbd_mpc574x_ec_toolbox/Communication Blocks/CAN Blocks/FCAN_Send  Priority=2  can_instance=0  can_mode=Non-blocking  can_timeout_ms=0  can_mb_idx=14  can_extended_id=off  can_is_remote=off  can_id=160  show_adv_opts=off  can_fd_enable=off  can_enable_brs=off  can_fd_padding=0
      settings: SourceProductName=NXP Model-Based Design Toolbox for MPC57xx MCUs
  VCU_BMS : canmsglib/CAN Pack  CANdbFile=D:\VCU\VCU_SL_ZhengZhou\ZT2\模型与接口\CAN_DBC\整车CANA_GBK.dbc  MsgList=(none)  MsgName=VCU_BMS  MsgIDType=Standard (11-bit identifier)  MsgIdentifier=352  MsgLength=8  SignalInfo=VCU_PowerOnReq$0$1$2$2$1$0$1$0$0$1$#VCU_UrgencyCutOffPowerReq$1$1$2$2$1$0$1$0$0$1$#  NSignals=2  StartBits=str2num('[int32(0);int32(1)]')  SignalSizes=str2num('[int32(1);int32(1)]')  ByteOrders=str2num('[int32(2);int32(2)]')  DataTypes=str2num('[int32(2);int32(2)]')  MultiplexTypes=str2num('[int32(1);int32(1)]')  MultiplexValues=str2num('[double(0);double(0)]')  Factors=str2num('[double(1);double(1)]')  Offsets=str2num('[double(0);double(0)]')  Minimums=str2num('[double(0);double(0)]')  Maximums=str2num('[double(1);double(1)]')  Remote=off  ApplyMinMax=off  BusOutput=on
      settings: SourceProductName=Simulink Real-Time  SourceProductBaseCode=XP  DataFormat=CANdb specified signals
  wires:
  VCU_BMS/1 -> Bus Selector/1
  Bus Selector/2 -> FCAN_Send_ID_0x160/2  "<Length>"
  Bus Selector/1 -> FCAN_Send_ID_0x160/1  "<Data>"
  Add/1 -> Data Store Write/1
  Data Store Read/1 -> Add/1
  Constant2/1 -> Add/2
  "BMS_OUT "/1 -> Bus Selector1/1
  Bus Selector1/1 -> ?  "<VCU_PowerOnReq>"
  Bus Selector1/2 -> ?  "<VCU_UrgencyCutOffPowerReq>"
  Data Type Conversion/1 -> VCU_BMS/1
  Data Type Conversion1/1 -> VCU_BMS/2
  Data Store Read1/1 -> Data Type Conversion/1
  Data Store Read2/1 -> Data Type Conversion1/1

== system ZT_VehCtrl_18B_CAN/SigOut/BRS ==
  "BRS_OUT " : Inport
  Trigger : TriggerPort  VariantControl=Variant  PortDimensions=1
  Add : Sum
  Bus Selector : BusSelector  OutputSignals=Data,Length
  Bus Selector1 : BusSelector  Commented=on  OutputSignals=MaxChargePowerLimit,OnOffCmd,BRS_PowerReq
  Constant : Constant  Value=0
  Constant1 : Constant  Value=0
  Constant4 : Constant  OutDataTypeStr=uint8
  Data Store Read : DataStoreRead  DataStoreName=Cnt_BRS_OUT
  Data Store Read1 : DataStoreRead  DataStoreName=Cnt_BRS_OUT
  Data Store Read4 : DataStoreRead  DataStoreName=OnOffCmd
  Data Store Write : DataStoreWrite  DataStoreName=Cnt_BRS_OUT
  Data Type Conversion : DataTypeConversion  OutDataTypeStr=single
  Data Type Conversion1 : DataTypeConversion  OutDataTypeStr=single
  Data Type Conversion2 : DataTypeConversion  OutDataTypeStr=boolean
  Data Type Conversion3 : DataTypeConversion  OutDataTypeStr=single
  FCAN_Send_ID_0x0CF109A7 : mbd_mpc574x_ec_toolbox/Communication Blocks/CAN Blocks/FCAN_Send  Priority=2  can_instance=0  can_mode=Non-blocking  can_timeout_ms=0  can_mb_idx=23  can_extended_id=on  can_is_remote=off  can_id=0CF109A7  show_adv_opts=off  can_fd_enable=off  can_enable_brs=off  can_fd_padding=0
      settings: SourceProductName=NXP Model-Based Design Toolbox for MPC57xx MCUs
  VCU2BRS : canmsglib/CAN Pack  CANdbFile=D:\VCU\VCU_SL_ZhengZhou\ZT2\模型与接口\CAN_DBC\整车CANA_GBK.dbc  MsgList=(none)  MsgName=VCU2BRS  MsgIDType=Extended (29-bit identifier)  MsgIdentifier=217123239  MsgLength=8  SignalInfo=LiveCounter$56$8$1$2$1$0$1$0$0$255$#MaxChargePowerLimit$16$16$1$2$1$0$1$0$0$500$#OnOffCmd$46$1$1$2$1$0$1$0$0$1$#PowerReq$0$16$1$2$1$0$1$0$0$500$#  NSignals=4  StartBits=str2num('[int32(56);int32(16);int32(46);int32(0)]')  SignalSizes=str2num('[int32(8);int32(16);int32(1);int32(16)]')  ByteOrders=str2num('[int32(1);int32(1);int32(1);int32(1)]')  DataTypes=str2num('[int32(2);int32(2);int32(2);int32(2)]')  MultiplexTypes=str2num('[int32(1);int32(1);int32(1);int32(1)]')  MultiplexValues=str2num('[double(0);double(0);double(0);double(0)]')  Factors=str2num('[double(1);double(1);double(1);double(1)]')  Offsets=str2num('[double(0);double(0);double(0);double(0)]')  Minimums=str2num('[double(0);double(0);double(0);double(0)]')  Maximums=str2num('[double(255);double(500);double(1);double(500)]')  Remote=off  ApplyMinMax=off  BusOutput=on
      settings: SourceProductName=Simulink Real-Time  SourceProductBaseCode=XP  DataFormat=CANdb specified signals
  wires:
  VCU2BRS/1 -> Bus Selector/1
  Bus Selector/1 -> FCAN_Send_ID_0x0CF109A7/1  "<Data>"
  Bus Selector/2 -> FCAN_Send_ID_0x0CF109A7/2  "<Length>"
  Add/1 -> Data Store Write/1
  Data Store Read/1 -> Add/1
  Constant4/1 -> Add/2
  Bus Selector1/3 -> ?  "<BRS_PowerReq>"
  Bus Selector1/1 -> ?  "<MaxChargePowerLimit>"
  "BRS_OUT "/1 -> Bus Selector1/1
  Bus Selector1/2 -> ?  "<OnOffCmd>"
  Data Type Conversion2/1 -> VCU2BRS/3
  Data Type Conversion/1 -> VCU2BRS/2
  Data Type Conversion1/1 -> VCU2BRS/4
  Data Store Read1/1 -> Data Type Conversion3/1
  Data Type Conversion3/1 -> VCU2BRS/1
  Data Store Read4/1 -> Data Type Conversion2/1
  Constant/1 -> Data Type Conversion/1
  Constant1/1 -> Data Type Conversion1/1

== system ZT_VehCtrl_18B_CAN/SigOut/DCDC ==
  "DCDC_OUT " : Inport
  Trigger : TriggerPort  VariantControl=Variant  PortDimensions=1
  Add : Sum
  Bus Selector : BusSelector  OutputSignals=Data,Length
  Bus Selector1 : BusSelector  Commented=on  OutputSignals=VCU_DCDC1_En
  Constant : Constant  OutDataTypeStr=uint8
  Data Store Read : DataStoreRead  DataStoreName=Cnt_DCDC_OUT
  Data Store Read5 : DataStoreRead  DataStoreName=VCU_DCDC1_En
  Data Store Write : DataStoreWrite  DataStoreName=Cnt_DCDC_OUT
  Data Type Conversion : DataTypeConversion  OutDataTypeStr=single
  FCAN_Send_ID_0x18008FD0 : mbd_mpc574x_ec_toolbox/Communication Blocks/CAN Blocks/FCAN_Send  Priority=2  can_instance=1  can_mode=Non-blocking  can_timeout_ms=0  can_mb_idx=47  can_extended_id=on  can_is_remote=off  can_id=18008FD0  show_adv_opts=off  can_fd_enable=off  can_enable_brs=off  can_fd_padding=0
      settings: SourceProductName=NXP Model-Based Design Toolbox for MPC57xx MCUs
  VCU_DCDC1 : canmsglib/CAN Pack  CANdbFile=D:\VCU\VCU_SL_ZhengZhou\ZT2\模型与接口\CAN_DBC\动力CANB_GBK.dbc  MsgList=(none)  MsgName=VCU_DCDC1  MsgIDType=Extended (29-bit identifier)  MsgIdentifier=402690000  MsgLength=8  SignalInfo=VCU_DCDC1_En$0$2$1$2$1$0$1$0$0$3$#  NSignals=1  StartBits=str2num('[int32(0)]')  SignalSizes=str2num('[int32(2)]')  ByteOrders=str2num('[int32(1)]')  DataTypes=str2num('[int32(2)]')  MultiplexTypes=str2num('[int32(1)]')  MultiplexValues=str2num('[double(0)]')  Factors=str2num('[double(1)]')  Offsets=str2num('[double(0)]')  Minimums=str2num('[double(0)]')  Maximums=str2num('[double(3)]')  Remote=off  ApplyMinMax=off  BusOutput=on
      settings: SourceProductName=Simulink Real-Time  SourceProductBaseCode=XP  DataFormat=CANdb specified signals
  wires:
  VCU_DCDC1/1 -> Bus Selector/1
  Bus Selector/2 -> FCAN_Send_ID_0x18008FD0/2  "<Length>"
  Bus Selector/1 -> FCAN_Send_ID_0x18008FD0/1  "<Data>"
  Add/1 -> Data Store Write/1
  Data Store Read/1 -> Add/1
  Constant/1 -> Add/2
  Data Type Conversion/1 -> VCU_DCDC1/1
  "DCDC_OUT "/1 -> Bus Selector1/1
  Bus Selector1/1 -> ?  "<VCU_DCDC1_En>"
  Data Store Read5/1 -> Data Type Conversion/1

== system ZT_VehCtrl_18B_CAN/SigOut/GPIO  ==
  note: LS
  note: PWM
  note: HS
  ETC : Subsystem
  HS : Subsystem
  PWM_OUT : Subsystem  Commented=on
  SPI0: LS09_14_15_16_1_2_11_4 : Subsystem
  SPI3: LS03_06_07_08_10_12_13_17_18_19 : Subsystem

== system ZT_VehCtrl_18B_CAN/SigOut/HVC ==
  "HVC_OUT " : Inport
  Trigger : TriggerPort  VariantControl=Variant  PortDimensions=1
  Add1 : Sum
  Bus Selector : BusSelector  OutputSignals=Data,Length
  Bus Selector1 : BusSelector  Commented=on  OutputSignals=EDrv1_PowOnCmd,EDrv2_PowOnCmd
  Constant6 : Constant  OutDataTypeStr=uint8
  Ctrl_HVC : canmsglib/CAN Pack  CANdbFile=D:\VCU\VCU_SL_ZhengZhou\ZT2\模型与接口\CAN_DBC\动力CANB_GBK.dbc  MsgList=(none)  MsgName=Ctrl_HVC  MsgIDType=Extended (29-bit identifier)  MsgIdentifier=402694405  MsgLength=8  SignalInfo=EDrv1_PowOnCmd$0$1$1$2$1$0$1$0$0$1$#EDrv2_PowOnCmd$2$1$1$2$1$0$1$0$0$1$#HvcCmd_Life$60$4$1$2$1$0$1$0$0$15$#PTC_PowOnCmd$6$1$1$2$1$0$1$0$0$1$#PaxAC_PowOnCmd$4$1$1$2$1$0$1$0$0$1$#  NSignals=5  StartBits=str2num('[int32(0);int32(2);int32(60);int32(6);int32(4)]')  SignalSizes=str2num('[int32(1);int32(1);int32(4);int32(1);int32(1)]')  ByteOrders=str2num('[int32(1);int32(1);int32(1);int32(1);int32(1)]')  DataTypes=str2num('[int32(2);int32(2);int32(2);int32(2);int32(2)]')  MultiplexTypes=str2num('[int32(1);int32(1);int32(1);int32(1);int32(1)]')  MultiplexValues=str2num('[double(0);double(0);double(0);double(0);double(0)]')  Factors=str2num('[double(1);double(1);double(1);double(1);double(1)]')  Offsets=str2num('[double(0);double(0);double(0);double(0);double(0)]')  Minimums=str2num('[double(0);double(0);double(0);double(0);double(0)]')  Maximums=str2num('[double(1);double(1);double(15);double(1);double(1)]')  Remote=off  ApplyMinMax=off  BusOutput=on
      settings: SourceProductName=Simulink Real-Time  SourceProductBaseCode=XP  DataFormat=CANdb specified signals
  Data Store Read : DataStoreRead  DataStoreName=Cnt_HVC_OUT
  Data Store Read1 : DataStoreRead  DataStoreName=Cnt_HVC_OUT
  Data Store Read6 : DataStoreRead  DataStoreName=EDrv1_PowOnCmd
  Data Store Read7 : DataStoreRead  DataStoreName=EDrv2_PowOnCmd
  Data Store Read8 : DataStoreRead  DataStoreName=PaxAC_PowOnCmd
  Data Store Read9 : DataStoreRead  DataStoreName=PTC_PowOnCmd
  Data Store Write1 : DataStoreWrite  DataStoreName=Cnt_HVC_OUT
  Data Type Conversion{,1..3} (4 alike) : DataTypeConversion  OutDataTypeStr=boolean
  Data Type Conversion15 : DataTypeConversion  OutDataTypeStr=single
  FCAN_Send_ID_0x1800A105 : mbd_mpc574x_ec_toolbox/Communication Blocks/CAN Blocks/FCAN_Send  Priority=2  can_instance=1  can_mode=Non-blocking  can_timeout_ms=0  can_mb_idx=48  can_extended_id=on  can_is_remote=off  can_id=1800A105  show_adv_opts=off  can_fd_enable=off  can_enable_brs=off  can_fd_padding=0
      settings: SourceProductName=NXP Model-Based Design Toolbox for MPC57xx MCUs
  wires:
  Bus Selector/1 -> FCAN_Send_ID_0x1800A105/1  "<Data>"
  Bus Selector/2 -> FCAN_Send_ID_0x1800A105/2  "<Length>"
  Ctrl_HVC/1 -> Bus Selector/1
  Add1/1 -> Data Store Write1/1
  Data Store Read1/1 -> Add1/1
  Constant6/1 -> Add1/2
  "HVC_OUT "/1 -> Bus Selector1/1
  Bus Selector1/1 -> ?  "<EDrv1_PowOnCmd>"
  Bus Selector1/2 -> ?  "<EDrv2_PowOnCmd>"
  Data Store Read/1 -> Data Type Conversion15/1
  Data Type Conversion15/1 -> Ctrl_HVC/3
  Data Type Conversion1/1 -> Ctrl_HVC/4
  Data Store Read9/1 -> Data Type Conversion1/1
  Data Store Read8/1 -> Data Type Conversion2/1
  Data Type Conversion2/1 -> Ctrl_HVC/5
  Data Store Read6/1 -> Data Type Conversion/1
  Data Type Conversion/1 -> Ctrl_HVC/1
  Data Store Read7/1 -> Data Type Conversion3/1
  Data Type Conversion3/1 -> Ctrl_HVC/2
